simulink model "sens_spray_vision"  (R2026b)
settings: Solver=VariableStepAuto
values from neighbouring files (symbols this model uses):
  D = zeros(nx, ny, 'uint8')    [sens_lidar2d_fast.m]
  P = (P + P.')/2    [sens_nav_ekf.m]
undefined symbols (not defined in the file or in its folder): Ts
libraries: simulink x4
settings Model: Creator=aomar  LastModifiedBy=aomar

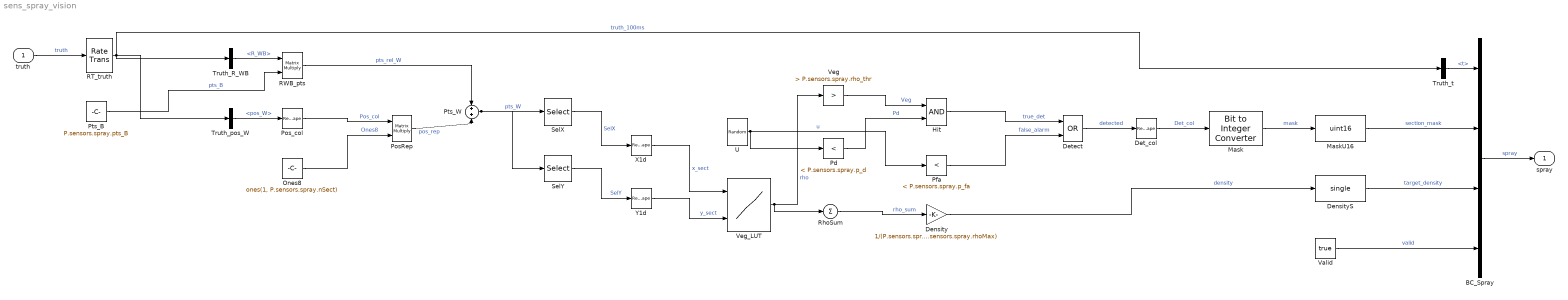
== system sens_spray_vision ==
  truth : Inport  OutDataTypeStr=Bus: Bus_TruthState  SampleTime=Ts.base
  BC_Spray : BusCreator  Inputs=4  OutDataTypeStr=Bus: Bus_SprayDemand  NonVirtualBus=on
      settings: InheritFromInputs=off
  Density : Gain  Gain=1/(P.sensors.spray.nSect*P.sensors.spray.rhoMax)
  DensityS : DataTypeConversion  OutDataTypeStr=single  RndMeth=Nearest  SaturateOnIntegerOverflow=off
  Det_col : Reshape  OutputDimensionality=Column vector (2-D)
  Detect : Logic  Operator=OR  AllPortsSameDT=off  OutDataTypeStr=boolean
  Hit : Logic  AllPortsSameDT=off  OutDataTypeStr=boolean
  Mask : simulink/Logic and Bit Operations/Bit to Integer Converter  nbits=P.sensors.spray.nSect  bitOrder=LSB first  signedOutputValues=Unsigned  outDtype=Inherit via internal rule  outDtypeSigned=Inherit via internal rule
      settings: LibrarySourceBlock=|
      | commutil2/Bit to Integer
      | Converter
  MaskU16 : DataTypeConversion  OutDataTypeStr=uint16  RndMeth=Nearest  SaturateOnIntegerOverflow=off
  Ones8 : Constant  Value=ones(1, P.sensors.spray.nSect)  VectorParams1D=off
  Pd : simulink/Logic and Bit Operations/Compare To Constant  relop=<  const=P.sensors.spray.p_d  OutDataTypeStr=boolean
  Pfa : simulink/Logic and Bit Operations/Compare To Constant  relop=<  const=P.sensors.spray.p_fa  OutDataTypeStr=boolean
  PosRep : Product  Multiplication=Matrix(*)
  Pos_col : Reshape  OutputDimensionality=Column vector (2-D)
  Pts_B : Constant  Value=P.sensors.spray.pts_B
  Pts_W : Sum
  RT_truth : RateTransition  OutPortSampleTime=Ts.spray
  RWB_pts : Product  Multiplication=Matrix(*)
  RhoSum : Sum  Inputs=+
  SelX : Selector  NumberOfDimensions=2  IndexOptions=Index vector (dialog),Select all  Indices=1,1  OutputSizes=1
  SelY : Selector  NumberOfDimensions=2  IndexOptions=Index vector (dialog),Select all  Indices=2,1  OutputSizes=1
  Truth_R_WB : BusSelector  OutputSignals=R_WB
  Truth_pos_W : BusSelector  OutputSignals=pos_W
  Truth_t : BusSelector  OutputSignals=t
  U : UniformRandomNumber  Minimum=zeros(1, P.sensors.spray.nSect)  Maximum=ones(1, P.sensors.spray.nSect)  Seed=P.sensors.spray.seeds  SampleTime=Ts.spray
  Valid : Constant  Value=true  OutDataTypeStr=boolean  SampleTime=Ts.spray
  Veg : simulink/Logic and Bit Operations/Compare To Constant  relop=>  const=P.sensors.spray.rho_thr  OutDataTypeStr=boolean
  Veg_LUT : Lookup_n-D  BreakpointsForDimension1=P.world.terrain.xE  BreakpointsForDimension2=P.world.terrain.yN  IndexSearchMethod=Evenly spaced points  Table=P.world.veg.rho  ExtrapMethod=Clip  InternalRulePriority=Speed  RndMeth=Simplest
      settings: InputPortMap=u0,u1
  X1d : Reshape
  Y1d : Reshape
  spray : Outport  OutDataTypeStr=Bus: Bus_SprayDemand
  wires:
  truth/1 -> RT_truth/1  "truth"
  Pts_B/1 -> RWB_pts/2  "pts_B"
  RT_truth/1 -> Truth_pos_W/1, Truth_t/1, Truth_R_WB/1  "truth_100ms"
  Truth_R_WB/1 -> RWB_pts/1  "<R_WB>"
  Truth_pos_W/1 -> Pos_col/1  "<pos_W>"
  RWB_pts/1 -> Pts_W/1  "pts_rel_W"
  Pos_col/1 -> PosRep/1  "Pos_col"
  Ones8/1 -> PosRep/2  "Ones8"
  PosRep/1 -> Pts_W/2  "pos_rep"
  Pts_W/1 -> SelY/1, SelX/1  "pts_W"
  SelX/1 -> X1d/1  "SelX"
  SelY/1 -> Y1d/1  "SelY"
  X1d/1 -> Veg_LUT/1  "x_sect"
  Y1d/1 -> Veg_LUT/2  "y_sect"
  U/1 -> Pfa/1, Pd/1  "u"
  Veg_LUT/1 -> Veg/1, RhoSum/1  "rho"
  RhoSum/1 -> Density/1  "rho_sum"
  Veg/1 -> Hit/1  "Veg"
  Pd/1 -> Hit/2  "Pd"
  Hit/1 -> Detect/1  "true_det"
  Pfa/1 -> Detect/2  "false_alarm"
  Density/1 -> DensityS/1  "density"
  Detect/1 -> Det_col/1  "detected"
  Det_col/1 -> Mask/1  "Det_col"
  Mask/1 -> MaskU16/1  "mask"
  Valid/1 -> BC_Spray/4  "valid"
  MaskU16/1 -> BC_Spray/2  "section_mask"
  DensityS/1 -> BC_Spray/3  "target_density"
  Truth_t/1 -> BC_Spray/1  "<t>"
  BC_Spray/1 -> spray/1  "spray"
